simulink model "PV_grid_LC_igbtmis"  (R2023a)
settings: Solver=FixedStepDiscrete  StartTime=0.0  StopTime=0.4  FixedStep=2.5e-07  RelTol=1e-3
undefined symbols (not defined in the file): Bias_i_val, C_val, fg_val, L_val, Lg_val, Rd_val, Rf_val, Rg_val, Ug_pk, Vdc_val
libraries: spsSeriesRLCBranchLib x4, spsVoltageMeasurementLib x4, spsCurrentMeasurementLib x3, spsUniversalBridgeLib x1, simulink x1, spsACVoltageSourceLib x1, spsDCVoltageSourceLib x1, spspowerguiLib x1
settings Model: Creator=35015  LastModifiedBy=35015

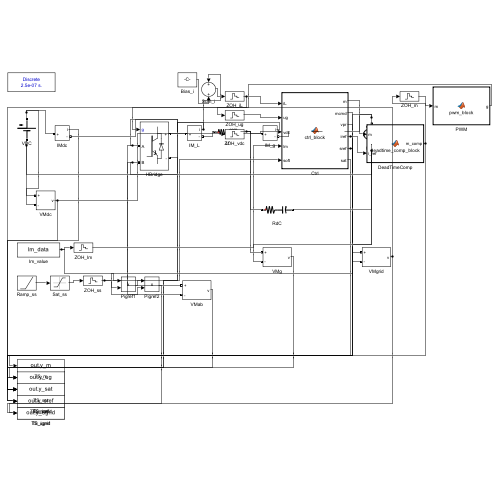
[thumbnail: Simulink's stored preview of the top-level diagram]
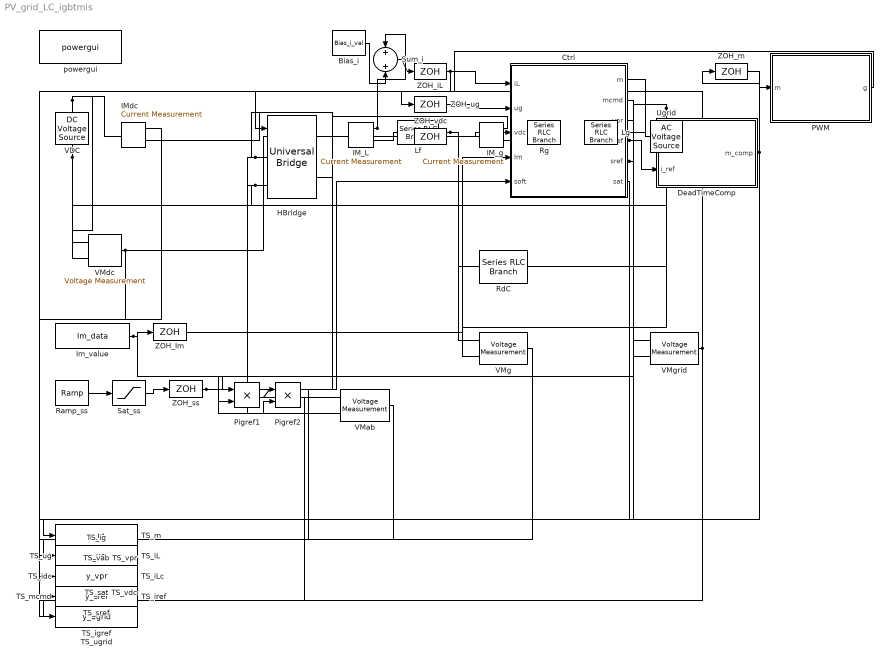
== system PV_grid_LC_igbtmis ==
  Bias_i : Constant  Value=Bias_i_val
  Ctrl : MATLAB Function  TreatAsAtomicUnit=on
  DeadTimeComp : MATLAB Function  TreatAsAtomicUnit=on
  HBridge : spsUniversalBridgeLib/Universal Bridge  Arms=2  SnubberResistance=1e5  SnubberCapacitance=inf  Device=IGBT / Diodes  Ron=Ron_sw  Lon=0  ForwardVoltages="[  0  0  ]"  ForwardVoltage=0  GTOparameters=[ 10e-6 , 20e-6 ]  IGBTparameters=[1e-7 2e-7]  Measurements=None  Measurements_2=None  converterType=Rectifier
  IM_L : spsCurrentMeasurementLib/Current Measurement  PhasorSimulation=off  OutputType=Complex  PSBequivalent=0
  IM_g : spsCurrentMeasurementLib/Current Measurement  PhasorSimulation=off  OutputType=Complex  PSBequivalent=0
  IMdc : spsCurrentMeasurementLib/Current Measurement  PhasorSimulation=off  OutputType=Complex  PSBequivalent=0
  Im_value : FromWorkspace  VariableName=Im_data  SampleTime=5e-05  Interpolate=off  OutputAfterFinalValue=Holding final value
  Lf : spsSeriesRLCBranchLib/Series RLC Branch  LConnTagsString=__new0  RConnTagsString=__new0  BranchType=RL  Resistance=Rf_val  Inductance=L_val  SetiL0=off  InitialCurrent=0  Capacitance=1e-6  Setx0=off  InitialVoltage=0  Measurements=None
  Lg : spsSeriesRLCBranchLib/Series RLC Branch  LConnTagsString=__new0  RConnTagsString=__new0  BranchType=RL  Resistance=0  Inductance=Lg_val  SetiL0=off  InitialCurrent=0  Capacitance=1e-6  Setx0=off  InitialVoltage=0  Measurements=None
  PWM : MATLAB Function  TreatAsAtomicUnit=on
  Pigref1 : Product
  Pigref2 : Product
  Ramp_ss : simulink/Sources/Ramp  slope=20  start=0  InitialOutput=0
  RdC : spsSeriesRLCBranchLib/Series RLC Branch  LConnTagsString=__new0  RConnTagsString=__new0  BranchType=RC  Resistance=Rd_val  Inductance=1e-3  SetiL0=off  InitialCurrent=0  Capacitance=C_val  Setx0=off  InitialVoltage=0  Measurements=None
  Rg : spsSeriesRLCBranchLib/Series RLC Branch  LConnTagsString=__new0  RConnTagsString=__new0  BranchType=R  Resistance=Rg_val  Inductance=1e-3  SetiL0=off  InitialCurrent=0  Capacitance=1e-6  Setx0=off  InitialVoltage=0  Measurements=None
  Sat_ss : Saturate  UpperLimit=1  LowerLimit=0
  Sum_i : Sum
  TS_iL : ToWorkspace  VariableName=y_iL  SaveFormat=Timeseries  SampleTime=-1
  TS_iLc : ToWorkspace  VariableName=y_iLc  SaveFormat=Timeseries  SampleTime=-1
  TS_idc : ToWorkspace  VariableName=y_idc  SaveFormat=Timeseries  SampleTime=-1
  TS_ig : ToWorkspace  VariableName=y_ig  SaveFormat=Timeseries  SampleTime=-1
  TS_igref : ToWorkspace  VariableName=y_igref  SaveFormat=Timeseries  SampleTime=-1
  TS_iref : ToWorkspace  VariableName=y_iref  SaveFormat=Timeseries  SampleTime=-1
  TS_m : ToWorkspace  VariableName=y_m  SaveFormat=Timeseries  SampleTime=-1
  TS_mcmd : ToWorkspace  VariableName=y_mcmd  SaveFormat=Timeseries  SampleTime=-1
  TS_sat : ToWorkspace  VariableName=y_sat  SaveFormat=Timeseries  SampleTime=-1
  TS_sref : ToWorkspace  VariableName=y_sref  SaveFormat=Timeseries  SampleTime=-1
  TS_ug : ToWorkspace  VariableName=y_ug  SaveFormat=Timeseries  SampleTime=-1
      settings: Decimation=20
  TS_ugrid : ToWorkspace  VariableName=y_ugrid  SaveFormat=Timeseries  SampleTime=-1
      settings: Decimation=20
  TS_vab : ToWorkspace  VariableName=y_vab  SaveFormat=Timeseries  SampleTime=-1
  TS_vdc : ToWorkspace  VariableName=y_vdc  SaveFormat=Timeseries  SampleTime=-1
      settings: Decimation=20
  TS_vpr : ToWorkspace  VariableName=y_vpr  SaveFormat=Timeseries  SampleTime=-1
  Ugrid : spsACVoltageSourceLib/AC Voltage Source  Amplitude=Ug_pk  Phase=0  Frequency=fg_val  SampleTime=0  Measurements=None  BusType=swing  Pref=10e3  Qref=0  Qmin=-inf  Qmax=+inf
  VDC : spsDCVoltageSourceLib/DC Voltage Source  Amplitude=Vdc_val  Measurements=None
  VMab : spsVoltageMeasurementLib/Voltage Measurement  PhasorSimulation=off  OutputType=Complex  PSBequivalent=0
  VMdc : spsVoltageMeasurementLib/Voltage Measurement  PhasorSimulation=off  OutputType=Complex  PSBequivalent=0
  VMg : spsVoltageMeasurementLib/Voltage Measurement  PhasorSimulation=off  OutputType=Complex  PSBequivalent=0
  VMgrid : spsVoltageMeasurementLib/Voltage Measurement  PhasorSimulation=off  OutputType=Complex  PSBequivalent=0
  ZOH_Im : ZeroOrderHold  SampleTime=5e-05
  ZOH_iL : ZeroOrderHold  SampleTime=5e-05
  ZOH_m : ZeroOrderHold  SampleTime=2.5e-07
  ZOH_ss : ZeroOrderHold  SampleTime=5e-05
  ZOH_ug : ZeroOrderHold  SampleTime=5e-05
  ZOH_vdc : ZeroOrderHold  SampleTime=5e-05
  powergui : spspowerguiLib/powergui  Priority=1  SimulationMode=Discrete  SampleTime=2.5e-07  frequency=50  Iterations=50  frequencyindice=60  Pbase=100e6  ErrMax=1e-4  UnitsV=kV  UnitsW=MW  buscounter=0  FunctionMessages=off  echomessages=off  EnableUseOfTLC=off  CurrentSourceSwitches=off  DisableSnubberDevices=off  DisableRonSwitches=off  DisableVfSwitches=off  DisplayEquations=off  AutomaticDiscreteSolvers=off  SolverType=Tustin/Backward Euler (TBE)  Interpol=off  ExternalGateDelay=off  methode=off  Ts=100  x0status=blocks  SPID=on  SwTol=0  HookPort=off  NonlinearTolerance=1e-4  nMaxIteration=100  ContinueOnMaxIteration=off  RestoreLinks=warning  ResistiveCurrentMeasurement=off  Frange=[0:2:500]  Ylog=off  Xlog=on  ShowGrid=off  save=off  variable=ZData  structure=0  ZoomFFT=off  StartTime=0.0  cycles=1  DisplayStyle=1  fundamental=60  FreqAxis=off  MaxFrequency=1000  frequencyindicesteady=1  RmsSteady=1  display=off
  wires:
  IM_L/1 -> Sum_i/1, TS_iL/1
  Bias_i/1 -> Sum_i/2
  VMdc/1 -> ZOH_vdc/1, TS_vdc/1
  Sum_i/1 -> ZOH_iL/1
  VMgrid/1 -> ZOH_ug/1, TS_ugrid/1
  Im_value/1 -> ZOH_Im/1, Pigref1/1
  Ramp_ss/1 -> Sat_ss/1
  Sat_ss/1 -> ZOH_ss/1
  ZOH_iL/1 -> Ctrl/1(iL), TS_iLc/1
  ZOH_ug/1 -> Ctrl/2(ug)
  ZOH_vdc/1 -> Ctrl/3(vdc)
  ZOH_Im/1 -> Ctrl/4(Im)
  ZOH_ss/1 -> Ctrl/5(soft), Pigref2/2
  Ctrl/5(sref) -> Pigref1/2, TS_sref/1
  Pigref1/1 -> Pigref2/1
  Pigref2/1 -> TS_igref/1
  Ctrl/1(m) -> DeadTimeComp/1(m)
  Ctrl/4(iref) -> DeadTimeComp/2(i_ref), TS_iref/1
  DeadTimeComp/1(m_comp) -> ZOH_m/1, TS_m/1
  ZOH_m/1 -> PWM/1(m)
  PWM/1(g) -> HBridge/1
  IM_g/1 -> TS_ig/1
  VMg/1 -> TS_ug/1
  VMab/1 -> TS_vab/1
  IMdc/1 -> TS_idc/1
  Ctrl/2(mcmd) -> TS_mcmd/1
  Ctrl/3(vpr) -> TS_vpr/1
  Ctrl/6(sat) -> TS_sat/1
  connections:
  IMdc/LConn1 -- VDC/RConn1 -- VMdc/LConn1
  IMdc/RConn1 -- HBridge/RConn1
  HBridge/RConn2 -- VDC/LConn1 -- VMdc/LConn2
  IM_L/LConn1 -- HBridge/LConn1 -- VMab/LConn1
  IM_L/RConn1 -- Lf/LConn1
  IM_g/LConn1 -- Lf/RConn1 -- VMg/LConn1 -- RdC/LConn1
  IM_g/RConn1 -- Rg/LConn1
  Rg/RConn1 -- Lg/LConn1
  Ugrid/RConn1 -- Lg/RConn1 -- VMgrid/LConn1
  HBridge/LConn2 -- Ugrid/LConn1 -- VMg/LConn2 -- VMgrid/LConn2 -- RdC/RConn1 -- VMab/LConn2

== matlab function PV_grid_LC_igbtmis/DeadTimeComp ==
  data: m input; m_comp output; i_ref input
function m_comp = deadtime_comp_block(m,i_ref)
%#codegen
cfg = deadtime_comp_mis_cfg();
m_comp = deadtime_comp_step(m,i_ref,cfg);
end

== matlab function PV_grid_LC_igbtmis/Ctrl ==
  data: iL input; m output; ug input; vdc input; Im input; soft input; mcmd output; vpr output; iref output; sref output; sat output
function [m,mcmd,vpr,iref,sref,sat] = ctrl_block(iL,ug,vdc,Im,soft)
%#codegen
[m,mcmd,vpr,iref,sref,sat] = ctrl_step_LC(iL,ug,vdc,Im,soft);
end

== matlab function PV_grid_LC_igbtmis/PWM ==
  data: m input; g output
function g = pwm_block(m)
%#codegen
persistent st
if isempty(st), st = pwm_init(); end
cfg = struct('Ts',2.4999999999999999e-07,'Tsw',5.0000000000000002e-05,'Nd',4);
[g,st] = pwm_bipolar(m,st,cfg);
end
